simulink model "Simulation"  (R2026b)
settings: Solver=VariableStepAuto  StopTime=20.0
settings Model: Creator=adelepinheirost-pierre  LastModifiedBy=adelepinheirost-pierre

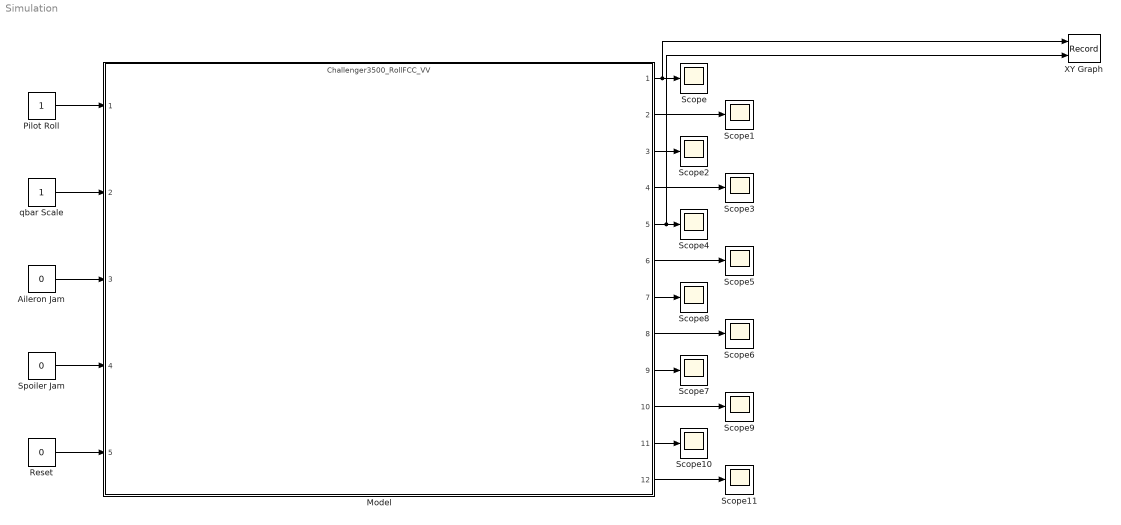
== system Simulation ==
  Aileron Jam : Constant  Value=0
  Model : ModelReference  ModelNameDialog=Challenger3500_RollFCC_VV  SimulationMode=Normal  ModelReferenceVersion=1.2
  Pilot Roll : Constant
  Reset : Constant  Value=0
  Scope{,1..11} (12 alike) : Scope
      Scope settings: ActiveDisplayYMinimum=13.089513070667492  ActiveDisplayYMaximum=25.440891299525653
      Scope1 settings: ActiveDisplayYMinimum=15.056046698139879  ActiveDisplayYMaximum=27.073385785245407
      Scope10 settings: DataLoggingVariableName=ScopeData10
      Scope11 settings: DataLoggingVariableName=ScopeData11
      Scope2 settings: DataLoggingVariableName=ScopeData2
      Scope3 settings: DataLoggingVariableName=ScopeData3
      Scope4 settings: DataLoggingVariableName=ScopeData4
      Scope5 settings: DataLoggingVariableName=ScopeData5
      Scope6 settings: ActiveDisplayYMinimum=-19.692020048894754  ActiveDisplayYMaximum=121.59510740996052  DataLoggingVariableName=ScopeData6
      Scope7 settings: ActiveDisplayYMinimum=-487.2277273819995  ActiveDisplayYMaximum=4975.6286099313293  DataLoggingVariableName=ScopeData7
      Scope8 settings: DataLoggingVariableName=ScopeData8
      Scope9 settings: DataLoggingVariableName=ScopeData9
  Spoiler Jam : Constant  Value=0
  XY Graph : Record  NumPorts=2.0  FileSettingsInternal="{\"entries\":[{\"content\":{\"excelSettings\":{\"content\":{},\"type\":\"Streamout.ExcelSettings\"},\"parquetSettings\":{\"content\":{},\"type\":\"Streamout.ParquetSettings\"}},\"type\":\"Streamout.FileSettingStorage\",\"uuid\":\"\"}],\"packageUris\":[\"http:\\/\\/schema.mathworks.com\\/mf0\\/streamout_blocks\\/R2020a\"],\"version\":\"1.0\"}"  FrameSettings=[0, 0]  Layout=[1 1]  SignalsInternal="{\"entries\":[{\"content\":{\"signals\":[{\"content\":{\"blockPath\":[],\"dimensions\":[1],\"domain\":\"\",\"lineColor\":\"#a2142f\",\"plots\":[ 1 ],\"port\":1,\"sid\":[\"\"],\"signalID\":1,\"signalName\":\"Model:1\"},\"type\":\"RecordBlkView.Signal\",\"uuid\":\"\"},{\"content\":{\"blockPath\":[],\"dimensions\":[1],\"domain\":\"\",\"lineColor\":\"#139fff\",\"plots\":[ 1 ],\"port\":2,\"sid\":[\"\"],\"signalID\":2,\"signalName\":\"Model:5\"},\"type\":\"RecordBlkView.Signal\",\"uuid\":\"\"}]},\"type\":\"RecordBlkView.InputSignals\",\"uuid\":\"\"}],\"packageUris\":[\"http:\\/\\/schema.mathworks.com\\/mf0\\/streamout_blocks\\/R2020a\"],\"version\":\"1.0\"}"  VisualizationBindings="{\"xyplotplugin\":{\"info\":[{\"series\":[{\"bindingParametersList\":[{\"parameter\":\"X-Axis\",\"signalID\":1,\"signalName\":\"Model:1\"},{\"parameter\":\"Y-Axis\",\"signalID\":2,\"signalName\":\"Model:5\"}],\"seriesID\":0}],\"subplotID\":1}]}}"  CompatibilityTag=XY
  qbar Scale : Constant
  wires:
  Pilot Roll/1 -> Model/1
  qbar Scale/1 -> Model/2
  Aileron Jam/1 -> Model/3
  Spoiler Jam/1 -> Model/4
  Reset/1 -> Model/5
  Model/1 -> XY Graph/1, Scope/1
  Model/2 -> Scope1/1
  Model/3 -> Scope2/1
  Model/4 -> Scope3/1
  Model/5 -> XY Graph/2, Scope4/1
  Model/6 -> Scope5/1
  Model/7 -> Scope8/1
  Model/8 -> Scope6/1
  Model/9 -> Scope7/1
  Model/10 -> Scope9/1
  Model/11 -> Scope10/1
  Model/12 -> Scope11/1
